simulink model "FullFMS_SIM_V0_1_3_R2026a"  (R2026a)
settings: Solver=FixedStepAuto  StopTime=inf  FixedStep=0.01  MaxStep=0.01  RelTol=1e-2
PreLoadFcn:
  | load("BUS_CONFIG_SIM.mat"); run("Param_SIM_V0_1_3.m")
libraries: opcualib x8
(part 2 of 2)

== stateflow chart FullFMS_SIM_V0_1_3_R2026a/Chart_SIM ==
  settings: updateMethod=DISCRETE  sampleTime=Ts_SIM
  state Conveyor29 [parallel]
    settings: executionOrder=1
    state Idle
      entry: SimSensors_20.SS_29_Cart_Stat=false; SimSensors_20.SS_29_Optic=false; SimSensors_20.SS_29_Cart_Next=false;
    state Arriving
      entry: SimSensors_20.SS_29_Cart_Next=true; SimActuators_20.SA_20_Conveyor=true; SimSensors_20.SS_20_Controler_On=true;
    state AtStop
      entry: SimSensors_20.SS_29_Cart_Next=false; SimSensors_20.SS_29_Count=true; SimSensors_20.SS_29_Cart_Stat=true; SimSensors_20.SS_29_Optic=true;
      PartOnCart=true; CartAt29=true; SimActuators_20.SA_20_Conveyor=false;
    state Delivered
      entry: SimSensors_20.SS_29_Count=false; SimControl_20.SC_29_CartDel=true; CRouteIn54=true; SimASi_50.SR_54_CRoute_In=true;
      during: SimSensors_20.SS_29_Optic = PartOnCart;
    state Leaving
      entry: SimControl_20.SC_29_CartDel=false; CRouteIn54=false; SimASi_50.SR_54_CRoute_In=false; CartAt29=false;
    (default) -> Idle
    Leaving -> Idle : after(t_leave,sec)
    Idle -> Arriving : [nCart < N_PARTS]
    Arriving -> AtStop : after(t_conv,sec)
    AtStop -> Delivered : after(T_CONV_T6,sec)
    Delivered -> Leaving : [SimASi_50.SR_54_CRoute_Out]
  state HD1_Ctrl [parallel]
    settings: executionOrder=2
    state Init
      entry: SimControl_50.SC_52_Profibus=true; SimControl_50.SC_55_PD_Sort=false; SimASi_50.SR_54_CRoute_Out=false;
      SimActuators_50.SA_50_Claw_Down=false; SimActuators_50.SA_50_Close_Claw=false; SimActuators_50.SA_50_Claw_2_Del=false; SimActuators_50.SA_50_Claw_2_Cart=false;
    state Ready
      entry: SimControl_50.SC_55_Initialization=true;
    state N1_StartMove
      entry: SimControl_50.SC_55_PD_Sort=false;
    state N2_LowerClaw
      entry: SimActuators_50.SA_50_Claw_Down=true;
    state N3_CloseClaw
      entry: SimActuators_50.SA_50_Close_Claw=true;
    state N3_Raise
      entry: SimActuators_50.SA_50_Claw_Down=false;
    state N4_Claw2Del
      entry: SimActuators_50.SA_50_Claw_2_Cart=false; SimActuators_50.SA_50_Claw_2_Del=true;
    state N5_LowerClaw2
      entry: SimActuators_50.SA_50_Claw_Down=true;
    state N6_Release
      entry: SimActuators_50.SA_50_Close_Claw=false;
    state N6_Raise
      entry: SimActuators_50.SA_50_Claw_Down=false;
    state N7_PDSort
      entry: SimControl_50.SC_55_PD_Sort=true;
    state N8_Claw2Cart
      entry: SimActuators_50.SA_50_Claw_2_Del=false; SimActuators_50.SA_50_Claw_2_Cart=true; Claw2CartCmd=true;
    state N9_CRouteOut
      entry: SimActuators_50.SA_50_Claw_2_Cart=false; Claw2CartCmd=false; SimASi_50.SR_54_CRoute_Out=true;
      exit: SimASi_50.SR_54_CRoute_Out=false; nCart = nCart + 1;
    (default) -> Init
    Init -> Ready : [SimSensors_50.SS_50_Claw_Cart && SimSensors_50.SS_50_Claw_High && ~SimSensors_50.SS_50_Part_in_Claw]
    N9_CRouteOut -> Ready : after(T_HD1_T1,sec)
    Ready -> N1_StartMove : [CRouteIn54 && CartAt29 && SimSensors_20.SS_29_Optic && ~SimSensors_60.SS_60_SPart]
    N1_StartMove -> N2_LowerClaw : [~SimControl_50.SC_55_PD_Sort && SimSensors_50.SS_50_Claw_Cart && SimSensors_50.SS_50_Claw_High && ~SimSensors_50.SS_50_Part_in_Claw]
    N2_LowerClaw -> N3_CloseClaw : [SimSensors_50.SS_50_Claw_Cart && SimSensors_50.SS_50_Claw_Low]
    N3_CloseClaw -> N3_Raise : [SimSensors_50.SS_50_Part_in_Claw]
    N3_Raise -> N4_Claw2Del : [SimSensors_50.SS_50_Claw_High && SimSensors_50.SS_50_Part_in_Claw && ~SimSensors_50.SS_50_Claw_Del]
    N4_Claw2Del -> N5_LowerClaw2 : [SimSensors_50.SS_50_Claw_Del && SimSensors_50.SS_50_Claw_High && SimSensors_50.SS_50_Part_in_Claw]
    N5_LowerClaw2 -> N6_Release : [SimSensors_50.SS_50_Claw_Del && SimSensors_50.SS_50_Claw_Low]
    N6_Release -> N6_Raise : [~SimSensors_50.SS_50_Part_in_Claw]
    N6_Raise -> N7_PDSort : [SimSensors_50.SS_50_Claw_Del && SimSensors_50.SS_50_Claw_High && ~SimSensors_50.SS_50_Part_in_Claw]
    N7_PDSort -> N8_Claw2Cart
    N8_Claw2Cart -> N9_CRouteOut : [SimSensors_50.SS_50_Claw_Cart]
  state HD1_Plant [parallel]
    settings: executionOrder=3
    state Vertical [parallel]
      settings: executionOrder=1
      state High
        entry: SimSensors_50.SS_50_Claw_High=true; SimSensors_50.SS_50_Claw_Low=false;
      state GoingDown
        entry: SimSensors_50.SS_50_Claw_High=false;
      state Low
        entry: SimSensors_50.SS_50_Claw_Low=true;
      state GoingUp
        entry: SimSensors_50.SS_50_Claw_Low=false;
      (default) -> High
      GoingUp -> High [order 1] : after(t_v_up,sec)
      High -> GoingDown : [SimActuators_50.SA_50_Claw_Down]
      GoingUp -> GoingDown [order 2] : [SimActuators_50.SA_50_Claw_Down]
      GoingDown -> Low [order 1] : after(t_v_down,sec)
      GoingDown -> GoingUp [order 2] : [~SimActuators_50.SA_50_Claw_Down]
      Low -> GoingUp : [~SimActuators_50.SA_50_Claw_Down]
    state Horizontal [parallel]
      settings: executionOrder=2
      state AtCart
        entry: SimSensors_50.SS_50_Claw_Cart=true; SimSensors_50.SS_50_Claw_Del=false;
      state ToDel
        entry: SimSensors_50.SS_50_Claw_Cart=false;
      state AtDel
        entry: SimSensors_50.SS_50_Claw_Del=true;
      state ToCart
        entry: SimSensors_50.SS_50_Claw_Del=false;
      (default) -> AtCart
      ToCart -> AtCart : after(t_h_cart,sec)
      AtCart -> ToDel : [SimActuators_50.SA_50_Claw_2_Del]
      ToDel -> AtDel : after(t_h_del,sec)
      AtDel -> ToCart : [SimActuators_50.SA_50_Claw_2_Cart]
    state Gripper [parallel]
      settings: executionOrder=3
      state Empty
        entry: SimSensors_50.SS_50_Part_in_Claw=false;
      state Gripping
      state Holding
        entry: SimSensors_50.SS_50_Part_in_Claw=true; PartOnCart=false;
      state Releasing
      (default) -> HD1_Plant.Gripper.Empty
      Releasing -> HD1_Plant.Gripper.Empty : after(t_grip,sec){SimSensors_60.SS_60_SPart = SimSensors_60.SS_60_SPart || SimSensors_50.SS_50_Claw_Del;}
      HD1_Plant.Gripper.Empty -> Gripping : [SimActuators_50.SA_50_Close_Claw && SimSensors_50.SS_50_Claw_Low && SimSensors_50.SS_50_Claw_Cart && PartOnCart]
      Gripping -> Holding : after(t_grip,sec)
      Holding -> Releasing : [~SimActuators_50.SA_50_Close_Claw && SimSensors_50.SS_50_Claw_Low]
  state SORT_Ctrl [parallel]
    entry: SimControl_60.SC_62_Profibus=false; SimControl_60.SC_65_Initialization=false; SimControl_60.SC_65_ID_1=false; SimControl_60.SC_65_ID_2=false; SimControl_60.SC_65_Part_Sorted=false;
    SimControl_60.SC_65_RBS_Output = (SORT_MODE == 1); SimControl_60.SC_65_RSB_Output = (SORT_MODE == 2); SimControl_60.SC_65_BRS_Output = (SORT_MODE == 3); SimControl_60.SC_65_BSR_Output = (SORT_MODE == 4); SimControl_60.SC_65_SRB_Output = (SORT_MODE == 5); SimControl_60.SC_65_SBR_Output = (SORT_MODE == 6);
    SimActuators_60.SA_60_Conveyor=false; SimActuators_60.SA_60_P1=false; SimActuators_60.SA_60_P2=false; SimActuators_60.SA_60_Identify=false; SimActuators_60.SA_61_Led_Start=false; SimActuators_60.SA_61_Led_Reset=false; SimActuators_60.SA_61_Led_Extra1=false; SimActuators_60.SA_61_Led_Extra2=false; SimActuators_60.SA_61_Panel_O4=false; SimActuators_60.SA_61_Panel_O5=false; SimActuators_60.SA_61_Panel_O6=false; SimActuators_60.SA_61_Panel_O7=false;
    FBSel = (SORT_MODE == 1 && SimControl_60.SC_65_RBS_Output) || (SORT_MODE == 2 && SimControl_60.SC_65_RSB_Output) || (SORT_MODE == 3 && SimControl_60.SC_65_BRS_Output) || (SORT_MODE == 4 && SimControl_60.SC_65_BSR_Output) || (SORT_MODE == 5 && SimControl_60.SC_65_SRB_Output) || (SORT_MODE == 6 && SimControl_60.SC_65_SBR_Output);
    settings: executionOrder=4
    state FB1_Init [parallel]
      settings: executionOrder=1
      state FB1_N2_Check
        entry: SimControl_60.SC_62_Profibus=true; FB1Init=false; SimControl_60.SC_65_Initialization=false;
      state FB1_N3_ClearPart
        entry: FB1Conv=true; FB1IDPin=true;
      state FB1_N1_InitOk
        entry: FB1Init=true; SimControl_60.SC_65_Initialization=true;
      (default) -> FB1_N2_Check
      FB1_N3_ClearPart -> FB1_N2_Check : [FB1Conv && SimSensors_60.SS_60_Part_Pass]{FB1Conv=false; FB1IDPin=false;}
      FB1_N1_InitOk -> FB1_N2_Check : [SimSensors_60.SS_61_Reset]{FB1Conv=false; FB1IDPin=false; TrigConv=false; Lever1=false; Lever2=false; PinSort=false; PartDel=false;}
      FB1_N2_Check -> FB1_N1_InitOk [order 1] : [SimControl_60.SC_62_Profibus && ~FB1Conv && ~SimSensors_60.SS_60_SPart && ~SimSensors_60.SS_60_SInd && ~SimSensors_60.SS_60_SPhoto && ~SimSensors_60.SS_60_Part_Pass]
      FB1_N2_Check -> FB1_N3_ClearPart [order 2] : [SimSensors_60.SS_60_SPart || SimSensors_60.SS_60_SInd || SimSensors_60.SS_60_SPhoto]
    state FB4_9_Sort [parallel]
      settings: executionOrder=2
      state OB1_N4_9_Select
      state N1_StartConv
        entry: TrigConv=true; SimControl_60.SC_65_ID_1=false; SimControl_60.SC_65_ID_2=false;
      state N2_Identify
        en, du: if SimSensors_60.SS_60_SInd, SimControl_60.SC_65_ID_1=false; SimControl_60.SC_65_ID_2=true;
        elseif SimSensors_60.SS_60_SPhoto, SimControl_60.SC_65_ID_1=true; SimControl_60.SC_65_ID_2=true;
        else, SimControl_60.SC_65_ID_1=true; SimControl_60.SC_65_ID_2=false; end
      state N3_SelectLever
        entry: cID = 0;
        if SimControl_60.SC_65_ID_1 && SimControl_60.SC_65_ID_2, cID = 1; elseif SimControl_60.SC_65_ID_1, cID = 2; elseif SimControl_60.SC_65_ID_2, cID = 3; end
        Lever1 = (cID == SORT_MAP(SORT_MODE,1)); Lever2 = (cID == SORT_MAP(SORT_MODE,2)); PassStr = (cID == SORT_MAP(SORT_MODE,3));
        during: if (Lever1 && SimSensors_60.SS_60_SL1_Fwd) || (Lever2 && SimSensors_60.SS_60_SL2_Fwd) || (PassStr && SimSensors_60.SS_60_SL1_Bck && SimSensors_60.SS_60_SL2_Bck), PinSort = true; end
      state N4_PartDel
        entry: PartDel=true; Lever1=false;
        if SORT_MODE ~= 3, Lever2=false; end
      state N5_ResetNext
        entry: TrigConv=false; PinSort=false; PartDel=false; Lever1=false; Lever2=false; PassStr=false;
      (default) -> OB1_N4_9_Select
      N5_ResetNext -> OB1_N4_9_Select
      OB1_N4_9_Select -> N1_StartConv : [FB1Init && FBSel && SimControl_50.SC_55_PD_Sort && SimSensors_50.SS_50_Claw_Del]
      N1_StartConv -> N2_Identify
      N2_Identify -> N3_SelectLever : after(T_SORT_ID - Ts_SIM,sec)
      N3_SelectLever -> N4_PartDel : [SimSensors_60.SS_60_Part_Pass]
      N4_PartDel -> N5_ResetNext
    state OB1_N10_11 [parallel]
      settings: executionOrder=3
      state N10_Wait
        entry: SimControl_60.SC_65_Part_Sorted=false;
      state N10_PartPass
      state N11_PartSorted
        entry: SimControl_60.SC_65_Part_Sorted=true;
      (default) -> N10_Wait
      N11_PartSorted -> N10_Wait : after(T_SORT_T7,sec)
      N10_Wait -> N10_PartPass : [SimSensors_60.SS_60_Part_Pass]
      N10_PartPass -> N11_PartSorted : [~SimSensors_60.SS_60_Part_Pass]
    state FB3_Actuators [parallel]
      settings: executionOrder=4
      state FB3_Map
        during: ConvOn60 = SimSensors_60.SS_61_Key_Pos && (TrigConv || FB1Conv); SimActuators_60.SA_60_Conveyor = ConvOn60;
        SimActuators_60.SA_60_P1 = SimSensors_60.SS_61_Key_Pos && Lever1; SimActuators_60.SA_60_P2 = SimSensors_60.SS_61_Key_Pos && Lever2;
        SimActuators_60.SA_60_Identify = SimSensors_60.SS_61_Key_Pos && (PinSort || FB1IDPin);
        SimActuators_60.SA_61_Led_Start = SimSensors_60.SS_61_Key_Pos && FB1Init; SimActuators_60.SA_61_Led_Reset = SimSensors_60.SS_61_Key_Pos && SimSensors_60.SS_61_Reset;
        SimActuators_60.SA_61_Led_Extra1 = SimControl_60.SC_65_Part_Sorted; SimActuators_60.SA_61_Led_Extra2 = false;
        SimActuators_60.SA_61_Panel_O4 = false; SimActuators_60.SA_61_Panel_O5 = false; SimActuators_60.SA_61_Panel_O6 = false; SimActuators_60.SA_61_Panel_O7 = false;
      (default) -> SORT_Ctrl.FB3_Actuators.FB3_Map
  state SORT_Plant [parallel]
    entry: SimSensors_60.SS_60_SPart=false; SimSensors_60.SS_60_SInd=false; SimSensors_60.SS_60_SPhoto=false; SimSensors_60.SS_60_Part_Pass=false;
    SimSensors_60.SS_60_SL1_Bck=true; SimSensors_60.SS_60_SL1_Fwd=false; SimSensors_60.SS_60_SL2_Bck=true; SimSensors_60.SS_60_SL2_Fwd=false;
    SimSensors_60.SS_61_Key_Pos=true; SimSensors_60.SS_61_Start=false; SimSensors_60.SS_61_Stop=false; SimSensors_60.SS_61_Reset=false;
    SimSensors_60.SS_61_Panel_I4=false; SimSensors_60.SS_61_Panel_I5=false; SimSensors_60.SS_61_Panel_I6=false; SimSensors_60.SS_61_Panel_I7=false;
    settings: executionOrder=5
    state Part [parallel]
      settings: executionOrder=1
      state Empty
        entry: SimSensors_60.SS_60_Part_Pass=false;
      state AtEntry
        entry: sortColor = PART_COLORS(min(nSortIn+1, numel(PART_COLORS))); nSortIn = nSortIn + 1;
      state ToStopper
        entry: xSort = 0;
        during: if ConvOn60, xSort = xSort + Ts_SIM; end
        SimSensors_60.SS_60_SPart = xSort < t_s_spart_off;
        if xSort >= t_s_photo, SimSensors_60.SS_60_SPhoto = (sortColor ~= 2); end
        if xSort >= t_s_ind, SimSensors_60.SS_60_SInd = (sortColor == 3); end
      state AtStopper
      state Released
        entry: xSort = 0;
        if SimSensors_60.SS_60_SL1_Fwd, sortExit = 1; elseif SimSensors_60.SS_60_SL2_Fwd, sortExit = 2; else, sortExit = 3; end
        during: if ConvOn60, xSort = xSort + Ts_SIM; end
        if xSort >= t_s_ind_off, SimSensors_60.SS_60_SInd = false; end
        if xSort >= t_s_photo_off, SimSensors_60.SS_60_SPhoto = false; end
      state PartPass
        entry: SimSensors_60.SS_60_Part_Pass = true; SimSensors_60.SS_60_SInd = false; SimSensors_60.SS_60_SPhoto = false; nDone = nDone + 1;
      (default) -> SORT_Plant.Part.Empty
      PartPass -> SORT_Plant.Part.Empty : after(t_s_pp,sec)
      SORT_Plant.Part.Empty -> AtEntry : [SimSensors_60.SS_60_SPart]
      AtEntry -> ToStopper : [SimActuators_60.SA_60_Conveyor]
      ToStopper -> AtStopper : [xSort >= t_s_ind]
      AtStopper -> Released : [SimActuators_60.SA_60_Identify && SimActuators_60.SA_60_Conveyor]
      Released -> PartPass : [(sortExit == 1 && xSort >= t_s_pass1) || (sortExit == 2 && xSort >= t_s_pass2) || (sortExit == 3 && xSort >= t_s_pass3)]
    state Lever1 [parallel]
      settings: executionOrder=2
      state SL1_Bck
        entry: SimSensors_60.SS_60_SL1_Bck=true; SimSensors_60.SS_60_SL1_Fwd=false;
      state SL1_ToFwd
        entry: SimSensors_60.SS_60_SL1_Bck=false;
      state SL1_Fwd
        entry: SimSensors_60.SS_60_SL1_Fwd=true;
      state SL1_ToBck
        entry: SimSensors_60.SS_60_SL1_Fwd=false;
      (default) -> SL1_Bck
      SL1_ToBck -> SL1_Bck [order 1] : after(t_sl1_bck,sec)
      SL1_Bck -> SL1_ToFwd : [SimActuators_60.SA_60_P1]
      SL1_ToBck -> SL1_ToFwd [order 2] : [SimActuators_60.SA_60_P1]
      SL1_ToFwd -> SL1_Fwd [order 1] : after(t_sl1_fwd,sec)
      SL1_ToFwd -> SL1_ToBck [order 2] : [~SimActuators_60.SA_60_P1]
      SL1_Fwd -> SL1_ToBck : [~SimActuators_60.SA_60_P1]
    state Lever2 [parallel]
      settings: executionOrder=3
      state SL2_Bck
        entry: SimSensors_60.SS_60_SL2_Bck=true; SimSensors_60.SS_60_SL2_Fwd=false;
      state SL2_ToFwd
        entry: SimSensors_60.SS_60_SL2_Bck=false;
      state SL2_Fwd
        entry: SimSensors_60.SS_60_SL2_Fwd=true;
      state SL2_ToBck
        entry: SimSensors_60.SS_60_SL2_Fwd=false;
      (default) -> SL2_Bck
      SL2_ToBck -> SL2_Bck [order 1] : after(t_sl2_bck,sec)
      SL2_Bck -> SL2_ToFwd : [SimActuators_60.SA_60_P2]
      SL2_ToBck -> SL2_ToFwd [order 2] : [SimActuators_60.SA_60_P2]
      SL2_ToFwd -> SL2_Fwd [order 1] : after(t_sl2_fwd,sec)
      SL2_ToFwd -> SL2_ToBck [order 2] : [~SimActuators_60.SA_60_P2]
      SL2_Fwd -> SL2_ToBck : [~SimActuators_60.SA_60_P2]
  state TEST_Ctrl [parallel]
    entry: SimControl_70.SC_72_Profibus=false; SimControl_70.SC_75_Initialization=false; SimControl_70.SC_75_RQ_Delivery1=false; SimControl_70.SC_75_ID_Delivery1=false; SimControl_70.SC_75_RQ_Delivery2=false; SimControl_70.SC_75_ID_Delivery2=false; SimControl_70.SC_75_Part_Del=false; SimControl_70.SC_75_RQ_Part_Del=false; SimControl_70.SC_75_RQ_Wrong=false;
    SimControl_70.SC_75_Identified = (TEST_MODE == 1); SimControl_70.SC_75_Requested = (TEST_MODE == 2); SimControl_70.SC_75_Identified80 = (TEST_MODE == 1); SimControl_70.SC_75_Requested80 = (TEST_MODE == 2);
    SimActuators_70.SA_70_Elev_Down=false; SimActuators_70.SA_70_Elev_Up=false; SimActuators_70.SA_70_Eject_Part=false; SimActuators_70.SA_70_Air_On=false; SimActuators_70.SA_71_Led_Start=false; SimActuators_70.SA_71_Led_Reset=false; SimActuators_70.SA_71_Led_Extra1=false; SimActuators_70.SA_71_Led_Extra2=false; SimActuators_70.SA_71_Panel_O4=false; SimActuators_70.SA_71_Panel_O5=false; SimActuators_70.SA_71_Panel_O6=false; SimActuators_70.SA_71_Panel_O7=false;
    SimASi_70.SR_73_TestCartID=0; SimASi_70.SR_74_Request=false; SimASi_70.SR_74_No_Cart=true; SimASi_70.SR_74_Cart_Full=false; SimASi_70.SR_74_CRoute_Out=false; SimASi_70.SR_74_CRoute_In=false;
    settings: executionOrder=6
    state FB1_Init70 [parallel]
      settings: executionOrder=1
      state FB1_N2_N3_Check
        entry: SimControl_70.SC_72_Profibus=true; FB1Init70=false; SimControl_70.SC_75_Initialization=false;
        during: FB1ElevDown70 = ~ElevLow70;
      state FB1_N3_PistonPulse
        entry: FB1PistAdv70=true;
      state FB1_N1_N4_InitOk
        entry: FB1Init70=true; SimControl_70.SC_75_Initialization=true; FB1ElevDown70=false; FB1PistAdv70=false;
      (default) -> FB1_N2_N3_Check
      FB1_N3_PistonPulse -> FB1_N2_N3_Check : after(T_TEST_T1,sec){FB1PistAdv70=false;}
      FB1_N1_N4_InitOk -> FB1_N2_N3_Check : [SimSensors_70.SS_71_Reset]{IdenDel=false; IdenProc=false; EjectProc=false; ReturnElev=false; ReqDel=false; IdenColor=false; PartOk=false; EjectOk=false; PartDiff=false; EjectBad=false;}
      FB1_N2_N3_Check -> FB1_N1_N4_InitOk [order 1] : [~PartIn70 && ElevLow70 && PistBck70 && DIST_INIT_PROV == 1]
      FB1_N2_N3_Check -> FB1_N3_PistonPulse [order 2] : [ElevLow70 && PartIn70]
    state FB4_Identified [parallel]
      settings: executionOrder=2
      state OB1_N4_Off
      state FB4_Wait
      state N1_StartID
        entry: IdenDel=true; idA70=false; idB70=false; PartDel70=false; RQPartDel70=false;
      state N2_N3_Raise
        en, du: if PartIn70 && ElevLow70 && SInd70, idB70 = true; end
        FB4ElevUp = PartIn70 && PistBck70 && ArmMag80;
      state N4_Identify
        entry: IdenProc=true; FB4ElevUp=true;
        en, du: if ~idB70, idA70 = true; if Height70, idB70 = true; end; end
      state N5_EjectWaitCart
        entry: IdenProc=false; EjectProc=true; FB4ElevUp=true;
      state N5_EjectPush
        entry: FB4PistFwd=true; FB4Air=true;
      state N5_EjectEnd
        entry: FB4PistFwd=false; FB4Air=false;
        en, du: FB4CartFull = CartStat24 && Optic24 && ~PistBck24;
      state N6_ReturnElev
        entry: EjectProc=false; ReturnElev=true; FB4ElevUp=false; FB4CartFull=false; FB4ElevDown=ArmMag80;
      state N6_PartDel
        entry: FB4ElevDown=false; PartDel70=true; ReturnElev=false;
      (default) -> OB1_N4_Off
      OB1_N4_Off -> FB4_Wait : [FB1Init70 && SimControl_70.SC_75_Identified]
      N6_PartDel -> FB4_Wait
      FB4_Wait -> N1_StartID : [PartIn70]
      N1_StartID -> TEST_Ctrl.FB4_Identified.N2_N3_Raise
      TEST_Ctrl.FB4_Identified.N2_N3_Raise -> N4_Identify : [ElevHigh70 && FB4ElevUp]
      N4_Identify -> N5_EjectWaitCart : after(T_TEST_T2,sec)
      N5_EjectWaitCart -> N5_EjectPush : [~PistBck24 && CartStat24 && ~Optic24]
      N5_EjectPush -> N5_EjectEnd [order 1] : [Optic24]
      N5_EjectPush -> N5_EjectEnd [order 2] : after(T_TEST_T3,sec)
      N5_EjectEnd -> N6_ReturnElev : [PistBck70 && ~PartIn70 && Optic24]
      N6_ReturnElev -> N6_PartDel : [ElevLow70]
    state FB5_Requested [parallel]
      settings: executionOrder=3
      state OB1_N5_Off
      state FB5_Wait
      state N1_StartReq
        entry: ReqDel=true; PartDiff=false; idA70=false; idB70=false; PartDel70=false; RQPartDel70=false; RQWrong70=false;
      state N2_N3_Raise
        en, du: if PartIn70 && ElevLow70 && SInd70, idB70 = true; end
        FB5ElevUp = PartIn70 && PistBck70 && ArmMag80 && ~PartDiff;
      state N4_ColorWindow
        entry: IdenColor=true; FB5ElevUp=true;
        en, du: if ~idB70, idA70 = true; if Height70, idB70 = true; end; end
      state N4_ColorHold
      state N5_Compare
        entry: IdenColor=false; FB5ElevUp=false;
        if (idA70 == RQ1_70) && (idB70 == RQ2_70), PartOk=true; EjectOk=true;
        else, PartDiff=true; EjectBad=true; end
      state N6_EjectWaitCart
      state N6_EjectPush
        entry: FB5PistFwd1=true; FB5Air=true;
      state N6_EjectEnd
        entry: FB5PistFwd1=false; FB5Air=false;
        en, du: FB5CartFull = CartStat24 && Optic24 && ~PistBck24;
      state N7_ReturnElev
        entry: EjectOk=false; ReturnElev=true; FB5CartFull=false; FB5ElevDown1=ArmMag80;
      state N7_RQPartDel
        entry: FB5ElevDown1=false; RQPartDel70=true; ReturnElev=false; PartOk=false;
      state N10_ResetReq
        entry: ReqDel=false;
      state N8_DownBad
        entry: FB5ElevDown2=ArmMag80;
      state N8_EjectBad
        entry: FB5ElevDown2=false; FB5PistFwd2=true;
      state N8_WaitBack
        entry: FB5PistFwd2=false;
      state N9_RQWrong
        entry: EjectBad=false; RQWrong70=true;
      (default) -> OB1_N5_Off
      OB1_N5_Off -> FB5_Wait : [FB1Init70 && SimControl_70.SC_75_Requested]
      N10_ResetReq -> FB5_Wait
      N9_RQWrong -> FB5_Wait
      FB5_Wait -> N1_StartReq : [PartIn70]
      N1_StartReq -> TEST_Ctrl.FB5_Requested.N2_N3_Raise
      TEST_Ctrl.FB5_Requested.N2_N3_Raise -> N4_ColorWindow : [ElevHigh70 && FB5ElevUp]
      N4_ColorWindow -> N4_ColorHold : after(T_TEST_T8,sec)
      N4_ColorHold -> N5_Compare : after(T_TEST_T2 - T_TEST_T8,sec)
      N5_Compare -> N6_EjectWaitCart [order 1] : [PartOk]
      N5_Compare -> N8_DownBad [order 2] : [PartDiff]
      N6_EjectWaitCart -> N6_EjectPush : [~PistBck24 && CartStat24 && ~Optic24]
      N6_EjectPush -> N6_EjectEnd [order 1] : [Optic24]
      N6_EjectPush -> N6_EjectEnd [order 2] : after(T_TEST_T5,sec)
      N6_EjectEnd -> N7_ReturnElev : [PistBck70 && ~PartIn70 && Optic24]
      N7_ReturnElev -> N7_RQPartDel : [ElevLow70]
      N7_RQPartDel -> N10_ResetReq
      N8_DownBad -> N8_EjectBad : [ElevLow70]
      N8_EjectBad -> N8_WaitBack : after(T_TEST_T6,sec)
      N8_WaitBack -> N9_RQWrong : [PistBck70 && ~PartIn70]
    state OB1_N6_Routing [parallel]
      settings: executionOrder=4
      state OB1_N6_Wait
      state OB1_N6_T7_CRouteOut
        entry: SimASi_70.SR_74_CRoute_Out=true; RouteOut74=true;
      state OB1_N6_Hold
        entry: SimASi_70.SR_74_CRoute_Out=false; RouteOut74=false;
      (default) -> OB1_N6_Wait
      OB1_N6_Hold -> OB1_N6_Wait : [~PartDel70 && ~RQPartDel70]
      OB1_N6_Wait -> OB1_N6_T7_CRouteOut : [PartDel70 || RQPartDel70]
      OB1_N6_T7_CRouteOut -> OB1_N6_Hold : after(T_TEST_T7,sec)
    state FB3_OB1_Map [parallel]
      settings: executionOrder=5
      state FB3_Map
        during: ElevUp70 = KeyPos71 && (FB4ElevUp || FB5ElevUp);
        ElevDown70 = KeyPos71 && (FB1ElevDown70 || FB4ElevDown || FB5ElevDown1 || FB5ElevDown2);
        Eject70 = KeyPos71 && (FB1PistAdv70 || FB4PistFwd || FB5PistFwd1 || FB5PistFwd2);
        Air70 = KeyPos71 && (FB4Air || FB5Air);
        SimActuators_70.SA_70_Elev_Up = ElevUp70; SimActuators_70.SA_70_Elev_Down = ElevDown70; SimActuators_70.SA_70_Eject_Part = Eject70; SimActuators_70.SA_70_Air_On = Air70;
        NoCart74 = ~CartStat24; CartFull74 = (FB4CartFull && TEST_MODE == 1) || (FB5CartFull && TEST_MODE == 2) || (CartStat24 && Optic24);
        SimASi_70.SR_74_No_Cart = NoCart74; SimASi_70.SR_74_Cart_Full = CartFull74; CRouteIn80 = CRouteIn74;
        SimActuators_70.SA_71_Led_Start = KeyPos71 && FB1Init70; SimActuators_70.SA_71_Led_Extra1 = NoCart74; SimActuators_70.SA_71_Led_Extra2 = CartFull74;
        SimControl_70.SC_75_ID_Delivery1 = idA70; SimControl_70.SC_75_ID_Delivery2 = idB70; SimControl_70.SC_75_Part_Del = PartDel70;
        SimControl_70.SC_75_RQ_Part_Del = RQPartDel70; SimControl_70.SC_75_RQ_Wrong = RQWrong70;
      (default) -> TEST_Ctrl.FB3_OB1_Map.FB3_Map
  state TEST_Plant [parallel]
    entry: KeyPos71=true; ElevLow70=true; PistBck70=true;
    SimSensors_70.SS_71_Key_Pos=true; SimSensors_70.SS_71_Start=false; SimSensors_70.SS_71_Stop=false; SimSensors_70.SS_71_Reset=false;
    SimSensors_70.SS_71_Panel_I4=false; SimSensors_70.SS_71_Panel_I5=false; SimSensors_70.SS_71_Panel_I6=false; SimSensors_70.SS_71_Panel_I7=false;
    settings: executionOrder=7
    state Elevator [parallel]
      settings: executionOrder=1
      state Elev_Low
        entry: ElevLow70=true; ElevHigh70=false; SInd70 = PartIn70 && testColor == 3; SStation70=false;
      state Elev_GoingUp
        entry: tElev = 0;
        during: tElev = tElev + Ts_SIM; ElevLow70 = tElev < t_t_up_lowoff;
        SInd70 = (PartIn70 && testColor == 3 && tElev < t_t_metal_off) || (tElev >= t_t_up_ind && tElev < t_t_up_ind + 0.15);
        SStation70 = tElev >= t_t_up_sst && tElev < t_t_up_sst + 0.22;
        Height70 = PartIn70 && testColor ~= 2 && tElev >= t_t_up - t_t_height_pre;
      state Elev_High
        entry: ElevHigh70=true; ElevLow70=false; SInd70=false; SStation70=false; Height70 = PartIn70 && testColor ~= 2;
      state Elev_GoingDown
        entry: tElev = 0; Height70=false;
        during: tElev = tElev + Ts_SIM; ElevHigh70 = tElev < t_t_down_highoff;
        SStation70 = tElev >= t_t_down_sst && tElev < t_t_down_sst + 0.27;
        SInd70 = (tElev >= t_t_down_ind && tElev < t_t_down_ind + 0.18) || (PartIn70 && testColor == 3 && tElev >= t_t_down - 0.3);
      (default) -> Elev_Low
      Elev_GoingDown -> Elev_Low [order 1] : [tElev >= t_t_down]
      Elev_Low -> Elev_GoingUp : [ElevUp70 && ~ElevDown70]
      Elev_GoingDown -> Elev_GoingUp [order 2] : [ElevUp70 && ~ElevDown70]
      Elev_GoingUp -> Elev_High [order 1] : [tElev >= t_t_up]
      Elev_GoingUp -> Elev_GoingDown [order 2] : [ElevDown70]
      Elev_High -> Elev_GoingDown : [ElevDown70]
    state SlideToCart [parallel]
      settings: executionOrder=3
      state Slide_Empty
      state Slide_Moving
        entry: PartToCart=false;
      state Slide_OnCart
        entry: if CartStat24, SimSensors_20.SS_24_Optic=true; Optic24=true; CartHasPart=true; end
      (default) -> Slide_Empty
      Slide_OnCart -> Slide_Empty
      Slide_Empty -> Slide_Moving : [PartToCart]
      Slide_Moving -> Slide_OnCart : after(t_t_ej_cart - t_t_ej_spart,sec)
    state Sensors_Out [parallel]
      settings: executionOrder=4
      state S70_Map
        en, du: SimSensors_70.SS_70_SPart = PartIn70; SimSensors_70.SS_70_Elev_Low = ElevLow70; SimSensors_70.SS_70_Elev_High = ElevHigh70;
        SimSensors_70.SS_70_SInductive = SInd70; SimSensors_70.SS_70_SPart_Height = Height70; SimSensors_70.SS_70_Pist_Bck = PistBck70;
        SimSensors_70.SS_70_SStation = SStation70;
      (default) -> S70_Map
    state Piston [parallel]
      settings: executionOrder=2
      state Pist_Back
        entry: PistBck70=true;
      state Pist_Fwd
        entry: tPist = 0;
        during: tPist = tPist + Ts_SIM; PistBck70 = tPist < t_t_pist_fwd;
        if PartIn70 && tPist >= t_t_ej_spart
        PartIn70 = false; Height70 = false; SInd70 = false;
        if ElevHigh70, PartToCart = true; else, nReject = nReject + 1; end
        end
      state Pist_Return
        entry: PistBck70=false;
      (default) -> Pist_Back
      Pist_Return -> Pist_Back : after(t_t_pist_back,sec)
      Pist_Back -> Pist_Fwd : [Eject70]
      Pist_Fwd -> Pist_Return : [~Eject70]
  state Conveyor24 [parallel]
    settings: executionOrder=8
    state C24_Idle
      entry: SimSensors_20.SS_24_Cart_Stat=false; SimSensors_20.SS_24_Cart_Next=false; SimSensors_20.SS_24_Count=false; SimSensors_20.SS_24_Optic=false; SimSensors_20.SS_24_Pist_Bck=true;
      SimControl_20.SC_24_Request=false; SimControl_20.SC_24_CartDel=false; SimControl_20.SC_24_CRoute_In=false; SimControl_20.SC_24_CRoute_Out=false;
      CartStat24=false; Optic24=false; PistBck24=true; CartHasPart=false; CRouteIn74=false;
    state C24_Request
      entry: SimControl_20.SC_24_Request=true;
    state C24_Moving
      entry: SimControl_20.SC_24_Request=false;
    state C24_Count
      entry: SimSensors_20.SS_24_Count=true; SimSensors_20.SS_24_Cart_Next=true;
    state C24_N6_AtStop
      entry: SimSensors_20.SS_24_Count=false; SimSensors_20.SS_24_Cart_Next=false; SimSensors_20.SS_24_Cart_Stat=true; SimSensors_20.SS_24_Pist_Bck=false;
      CartStat24=true; PistBck24=false; SimControl_20.SC_24_CartDel=true; SimASi_70.SR_73_TestCartID = nTest + 1;
      RQ1_70 = RQ_DELIVERY(min(nTest + 1, size(RQ_DELIVERY,1)), 1) == 1; RQ2_70 = RQ_DELIVERY(min(nTest + 1, size(RQ_DELIVERY,1)), 2) == 1;
      SimControl_70.SC_75_RQ_Delivery1 = RQ1_70; SimControl_70.SC_75_RQ_Delivery2 = RQ2_70;
    state C24_CRouteIn
      entry: SimASi_70.SR_74_CRoute_In=true; SimControl_20.SC_24_CRoute_In=true; CRouteIn74=true;
    state C24_Docked
      entry: SimASi_70.SR_74_CRoute_In=false; SimControl_20.SC_24_CRoute_In=false; CRouteIn74=false;
    state C24_N7_CartDelOff
      entry: SimControl_20.SC_24_CartDel=false;
    state C24_Release
      entry: SimControl_20.SC_24_CRoute_Out=true;
    state C24_PinBack
      entry: SimSensors_20.SS_24_Pist_Bck=true; PistBck24=true;
    state C24_Leaving
      entry: SimSensors_20.SS_24_Optic=false; Optic24=false;
    state C24_Gone
      entry: SimSensors_20.SS_24_Cart_Stat=false; CartStat24=false; SimControl_20.SC_24_CRoute_Out=false;
      if CartHasPart, nTest = nTest + 1; end
    (default) -> C24_Idle
    C24_Gone -> C24_Idle
    C24_Idle -> C24_Request : [nTest < N_PARTS && FB1Init70]
    C24_Request -> C24_Moving : after(t_24_req,sec)
    C24_Moving -> C24_Count : after(t_24_arrive - t_24_req - t_24_count,sec)
    C24_Count -> C24_N6_AtStop : after(t_24_count,sec)
    C24_N6_AtStop -> C24_CRouteIn : after(t_24_croute_in0,sec)
    C24_CRouteIn -> C24_Docked : after(t_24_croute_in,sec)
    C24_Docked -> C24_N7_CartDelOff : after(T_CONV24_T1 - t_24_croute_in0 - t_24_croute_in,sec)
    C24_N7_CartDelOff -> C24_Release : [RouteOut74]
    C24_Release -> C24_PinBack : after(t_24_pist_bck,sec)
    C24_PinBack -> C24_Leaving : after(t_24_optic_off - t_24_pist_bck,sec)
    C24_Leaving -> C24_Gone : after(t_24_leave - t_24_optic_off,sec)
  state DIST_Feed_PROVISORIO [parallel]
    settings: executionOrder=9
    state DIST_Wait
      entry: ArmMag80=true;
    state DIST_ArmToStation
      entry: ArmMag80=false;
    state DIST_Drop
      entry: SStation70=true;
    state DIST_PartIn
      entry: PartIn70=true; testColor = PART_COLORS(min(nTestIn + 1, numel(PART_COLORS))); nTestIn = nTestIn + 1; SInd70 = (testColor == 3);
    state DIST_ArmBack
      entry: SStation70=false;
    (default) -> DIST_Wait
    DIST_ArmBack -> DIST_Wait : after(t_dist_arm - t_dist_sst_dur + t_dist_sst,sec)
    DIST_Wait -> DIST_ArmToStation : [(CRouteIn80 || RQWrong70) && ~PartIn70 && nTestIn < numel(PART_COLORS)]
    DIST_ArmToStation -> DIST_Drop : after(t_dist_feed - t_dist_sst,sec)
    DIST_Drop -> DIST_PartIn : after(t_dist_sst,sec)
    DIST_PartIn -> DIST_ArmBack : after(t_dist_sst_dur - t_dist_sst,sec)
  data: SimActuators_20 output Bus: B_SimActuators_20; SimControl_20 output Bus: B_SimControl_20; SimSensors_20 output Bus: B_SimSensors_20; SimActuators_50 output Bus: B_SimActuators_50; SimASi_50 output Bus: B_SimASi_50; SimControl_50 output Bus: B_SimControl_50; SimSensors_50 output Bus: B_SimSensors_50; SimActuators_60 output Bus: B_SimActuators_60; SimControl_60 output Bus: B_SimControl_60; SimSensors_60 output Bus: B_SimSensors_60; Ts_SIM parameter double; T_HD1_T1 parameter double; T_CONV_T6 parameter double; t_v_down parameter double; t_v_up parameter double; t_h_del parameter double; t_h_cart parameter double; t_grip parameter double; t_conv parameter double; t_leave parameter double; N_PARTS parameter double; SORT_MODE parameter double; T_SORT_ID parameter double; T_SORT_T7 parameter double; t_s_spart_off parameter double; t_s_photo parameter double; t_s_ind parameter double; t_s_ind_off parameter double; t_s_photo_off parameter double; t_s_pass1 parameter double; t_s_pass2 parameter double; t_s_pass3 parameter double; t_s_pp parameter double; t_sl1_fwd parameter double; t_sl1_bck parameter double; t_sl2_fwd parameter double; t_sl2_bck parameter double; PART_COLORS parameter double; SORT_MAP parameter double; PartOnCart local boolean =false; CartAt29 local boolean =false; CRouteIn54 local boolean =false; Claw2CartCmd local boolean =false; FB1Init local boolean =false; FB1Conv local boolean =false; FB1IDPin local boolean =false; FBSel local boolean =false; ConvOn60 local boolean =false; TrigConv local boolean =false; Lever1 local boolean =false; Lever2 local boolean =false; PassStr local boolean =false; PinSort local boolean =false; PartDel local boolean =false; nCart local double =0; nDone local double =0; nSortIn local double =0; sortColor local double =0; sortExit local double =0; cID local double =0; xSort local double =0; SimActuators_70 output Bus: B_SimActuators_70; SimASi_70 output Bus: B_SimASi_70; SimControl_70 output Bus: B_SimControl_70; SimSensors_70 output Bus: B_SimSensors_70; TEST_MODE parameter double; DIST_INIT_PROV parameter double; T_TEST_T1 parameter double; T_TEST_T2 parameter double; T_TEST_T8 parameter double; T_TEST_T3 parameter double; T_TEST_T5 parameter double; T_TEST_T6 parameter double; T_TEST_T7 parameter double; T_CONV24_T1 parameter double; t_t_up parameter double; t_t_up_lowoff parameter double; t_t_up_ind parameter double; t_t_up_sst parameter double; t_t_metal_off parameter double; t_t_height_pre parameter double; t_t_down parameter double; t_t_down_highoff parameter double; t_t_down_sst parameter double; t_t_down_ind parameter double; t_t_ej_spart parameter double; t_t_pist_fwd parameter double; t_t_pist_back parameter double; t_t_ej_cart parameter double; t_24_arrive parameter double; t_24_count parameter double; t_24_req parameter double; t_24_croute_in0 parameter double; t_24_croute_in parameter double; t_24_pist_bck parameter double; t_24_optic_off parameter double; t_24_leave parameter double; t_dist_feed parameter double; t_dist_sst parameter double; t_dist_sst_dur parameter double; t_dist_arm parameter double; RQ_DELIVERY parameter double; FB1Init70 local boolean =false; FB1ElevDown70 local boolean =false; FB1PistAdv70 local boolean =false; IdenDel local boolean =false; IdenProc local boolean =false; EjectProc local boolean =false; ReturnElev local boolean =false; FB4ElevUp local boolean =false; FB4ElevDown local boolean =false; FB4PistFwd local boolean =false; FB4Air local boolean =false; FB4CartFull local boolean =false; ReqDel local boolean =false; IdenColor local boolean =false; PartOk local boolean =false; EjectOk local boolean =false; PartDiff local boolean =false; EjectBad local boolean =false; FB5ElevUp local boolean =false; FB5ElevDown1 local boolean =false; FB5ElevDown2 local boolean =false; FB5PistFwd1 local boolean =false; FB5PistFwd2 local boolean =false; FB5Air local boolean =false; FB5CartFull local boolean =false; idA70 local boolean =false; idB70 local boolean =false; PartDel70 local boolean =false; RQPartDel70 local boolean =false; RQWrong70 local boolean =false; RQ1_70 local boolean =false; RQ2_70 local boolean =false; RouteOut74 local boolean =false; NoCart74 local boolean =false; CartFull74 local boolean =false; ElevUp70 local boolean =false; ElevDown70 local boolean =false; Eject70 local boolean =false; Air70 local boolean =false; CRouteIn80 local boolean =false; CRouteIn74 local boolean =false; CartStat24 local boolean =false; Optic24 local boolean =false; PistBck24 local boolean =false; ArmMag80 local boolean =false; KeyPos71 local boolean =false; PartToCart local boolean =false; CartHasPart local boolean =false; PartIn70 local boolean =false; ElevLow70 local boolean =false; ElevHigh70 local boolean =false; SInd70 local boolean =false; Height70 local boolean =false; PistBck70 local boolean =false; SStation70 local boolean =false; nTest local double =0; nTestIn local double =0; nReject local double =0; testColor local double =0; tElev local double =0; tPist local double =0
